simulink model "Firmware"  (R2024b)
settings: Solver=FixedStepDiscrete  StartTime=0.0  StopTime=34.5  FixedStep=0.001  RelTol=1e-3  EnableMultiTasking=on
PreLoadFcn:
  | startup;
  | createVariables;
undefined symbols (not defined in the file or in its folder): B, diff, eour6dof, ESP32, Levenberg, Marquardt, maxWaypoints, Spline, ts, waypointTimes, WROOM, X, Y, Z
libraries: sm_lib x46, nesl_utility x13, blocksLibrary x10, arduinolib x6, simulink_extras x6, robotcorelib x4, robotmaniplib x1, simulink x1
(part 1 of 2)
settings Model: PacingRate=10  ExtModeTrigDuration=2  Creator=esaro  LastModifiedBy=esaro
settings SolverCC: AutoInsertRateTranBlk=on
settings OptimizationCC: EnhancedBackFolding=on  PassReuseOutputArgsAs=Individual arguments  ZeroExternalMemoryAtStartup=off  ZeroInternalMemoryAtStartup=off  MaxStackSize=64  OptimizeBlockOrder=speed  DifferentSizesBufferReuse=on  OptimizationCustomize=off  EfficientTunableParamExpr=on
settings DebuggingCC: ParameterTunabilityLossMsg=error
settings HardwareCC: ProdBitPerPointer=32  ProdBitPerSizeT=32  ProdBitPerPtrDiffT=32  ProdLargestAtomicInteger=Long  ProdLargestAtomicFloat=Double  ProdWordSize=32  ProdHWDeviceType=ARM Compatible->ARM Cortex
settings SFSimCC: MATLABDynamicMemAlloc=off
settings RTWCC: Description=Embedded Coder  SystemTargetFile=ert.tlc  HardwareBoard=ESP32-WROOM(Arduino Compatible)  TLCOptions="-aInlineSetEventsForThisBaseRateFcn=TLC_FALSE -aSuppressMultiTaskScheduler=TLC_FALSE  -aRateBasedStepFcn=0"  TemplateMakefile=ert_default_tmf  Toolchain=ESP32  BuildConfiguration=Faster Runs
settings CodeAppCC: ForceParamTrailComments=on  IgnoreCustomStorageClasses=off  OperatorAnnotations=on  SimulinkDataObjDesc=on  SFDataObjDesc=on  InsertBlockDesc=on
settings ERTTargetCC: SupportContinuousTime=on  SupportVariableSizeSignals=on  ExtModeTransport=3  ExtModeStaticAlloc=on  ExtModeAutomaticAllocSize=off  ExtModeStaticAllocSize=65536  ExtModeMexFile=ext_xcp  ExtModeIntrfLevel=Level2 - Open  InlinedParameterPlacement=Hierarchical

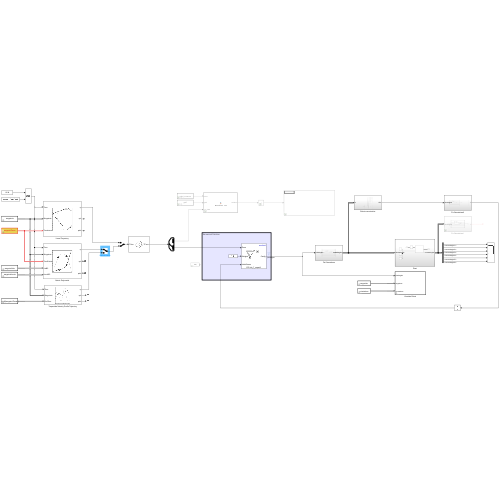
[thumbnail: Simulink's stored preview of the top-level diagram]
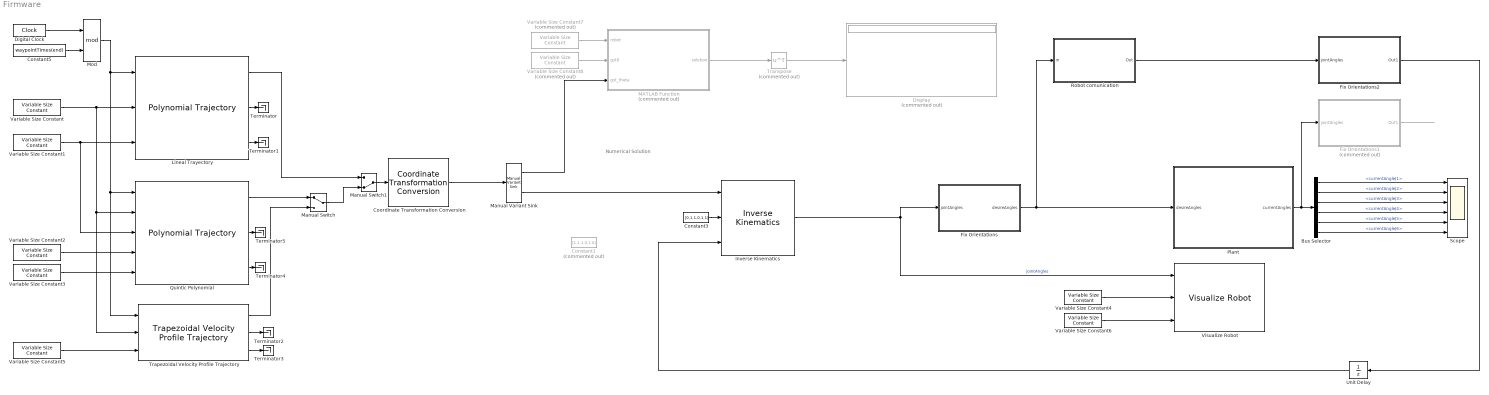
== system Firmware ==
  note: Numerical Solution
  Bus Selector : BusSelector  OutputSignals=currentAngleJ1,currentAngleJ2,currentAngleJ3,currentAngleJ4,currentAngleJ5,currentAngleJ6
  Constant1 : Constant  Commented=on  Value=[1,1,1,0,1,0]  VectorParams1D=off
  Constant3 : Constant  Value=[0,1,1,0,1,1]  VectorParams1D=off
  Constant5 : Constant  Value=waypointTimes(end)
  Coordinate Transformation Conversion : robotcorelib/Coordinate Transformation Conversion  InputRepresentation=Translation Vector  InputEulerSequence=ZYX  ShowTrVecInputPort=on  OutputRepresentation=Homogeneous Transformation  OutputEulerSequence=ZYX  ShowTrVecOutputPort=on  SimulateUsing=Interpreted execution
  Digital Clock : DigitalClock  SampleTime=ts
  Display : Display  Commented=on
  Fix Orientations : Subsystem
  Fix Orientations1 : Subsystem  Commented=on
  Fix Orientations2 : Subsystem
  Inverse Kinematics : robotmaniplib/Inverse Kinematics  RigidBodyTree=eour6dof  EndEffector=link_7_export2  ShowInfo=off  SolverName=Levenberg-Marquardt  EnforceJointLimits=on  MaxIterations=1500  MaxTime=10  GradientTolerance=1e-7  SolutionTolerance=1e-6  StepTolerance=1e-14  ErrorChangeTolerance=1e-12  UseErrorDamping=on  DampingBias=0.0025  SimulateUsing=Interpreted execution
  Lineal Trayectory : robotcorelib/Polynomial Trajectory  WaypointSource=External  Waypoints=[ 0, 2, 1, 5, 0; -1, 3, 1, 4, 4 ]  TimePoints=[ 0, 1, 2, 3, 4 ]  TimeInterval=[ 1, 4 ]  Method=B-Spline  ParameterSource=External  VelocityBoundaryCondition=zeros( 2, 5 )  AccelerationBoundaryCondition=zeros( 2, 5 )  SimulateUsing=Interpreted execution
  MATLAB Function : MATLAB Function  Commented=on  TreatAsAtomicUnit=on
  Manual Variant Sink : simulink/Signal Routing/Manual Variant Sink  NumChoices=2  LabelModeActiveChoice=V_2
  Manual Switch : ManualSwitch
  Manual Switch1 : ManualSwitch  CurrentSetting=0
  Mod : Math  Operator=mod  SignedPower=on
  Plant : Subsystem
  Quintic Polynomial : robotcorelib/Polynomial Trajectory  WaypointSource=External  Waypoints=[ 0, 2, 1, 5, 0; -1, 3, 1, 4, 4 ]  TimePoints=[ 0, 1, 2, 3, 4 ]  TimeInterval=[ 1, 4 ]  Method=Quintic Polynomial  ParameterSource=External  VelocityBoundaryCondition=zeros( 2, 5 )  AccelerationBoundaryCondition=zeros( 2, 5 )  SimulateUsing=Interpreted execution
  Robot comunication : Subsystem
  Scope : Scope  NumInputPorts=6
  Terminator{,1..5} (6 alike) : Terminator
  Transpose : Math  Commented=on  Operator=transpose
  Trapezoidal Velocity Profile Trajectory : robotcorelib/Trapezoidal Velocity Profile Trajectory  WaypointSource=External  Waypoints=[ 0, -0.5, -1; 0, 0.5, 1 ]  NumParams=1  Parameter1=End Time  Parameter2=End Time  ParameterSource=External  PeakVelocity=[ 1; 1; 1 ]  Acceleration=[ 1; 2 ]  EndTime=[ 1; 1; 1 ]  AccelTime=[ 1; 2 ]  SimulateUsing=Interpreted execution
  Unit Delay : UnitDelay  InitialCondition=ikInitGuess'  SampleTime=-1  HasFrameUpgradeWarning=on
  Variable Size Constant : blocksLibrary/Variable Size Constant  val=waypoints  maxSize=[3,maxWaypoints]  Ts=-1
  Variable Size Constant1 : blocksLibrary/Variable Size Constant  val=waypointTimes  maxSize=[1,maxWaypoints]  Ts=-1
  Variable Size Constant2 : blocksLibrary/Variable Size Constant  val=waypointVels  maxSize=[3,maxWaypoints]  Ts=-1
  Variable Size Constant3 : blocksLibrary/Variable Size Constant  val=waypointAccels  maxSize=[3,maxWaypoints]  Ts=-1
  Variable Size Constant4 : blocksLibrary/Variable Size Constant  val=waypoints  maxSize=[3,maxWaypoints]  Ts=-1
  Variable Size Constant5 : blocksLibrary/Variable Size Constant  val=repmat(diff(waypointTimes),[3 1])  maxSize=[3,maxWaypoints-1]  Ts=-1
  Variable Size Constant6 : blocksLibrary/Variable Size Constant  val=orientations  maxSize=[3,maxWaypoints]  Ts=-1
  Variable Size Constant7 : blocksLibrary/Variable Size Constant  Commented=on  val=robot_measure  maxSize=[4,1]  Ts=-1
  Variable Size Constant8 : blocksLibrary/Variable Size Constant  Commented=on  val=gst0  maxSize=[4,4]  Ts=-1
  Visualize Robot : blocksLibrary/Visualize Robot  rbtName=eour6dof  eeName=link_7_export2  numJoints=numel(eour6dof.homeConfiguration)  maxPts=maxWaypoints  plotMode=Trajectory
  wires:
  Bus Selector/1 -> Scope/1  "<currentAngleJ1>"
  Plant/1(currentAngles) -> Fix Orientations1/1(jointAngles), Bus Selector/1
  Constant3/1 -> Inverse Kinematics/2
  Bus Selector/4 -> Scope/4  "<currentAngleJ4>"
  Bus Selector/5 -> Scope/5  "<currentAngleJ5>"
  Bus Selector/6 -> Scope/6  "<currentAngleJ6>"
  Unit Delay/1 -> Inverse Kinematics/3
  Bus Selector/2 -> Scope/2  "<currentAngleJ2>"
  Digital Clock/1 -> Mod/1
  Constant5/1 -> Mod/2
  Trapezoidal Velocity Profile Trajectory/1 -> Manual Switch/2
  Trapezoidal Velocity Profile Trajectory/2 -> Terminator2/1
  Variable Size Constant3/1 -> Quintic Polynomial/5
  Variable Size Constant5/1 -> Trapezoidal Velocity Profile Trajectory/3
  Variable Size Constant2/1 -> Quintic Polynomial/4
  Lineal Trayectory/2 -> Terminator/1
  Trapezoidal Velocity Profile Trajectory/3 -> Terminator3/1
  Lineal Trayectory/3 -> Terminator1/1
  Variable Size Constant6/1 -> Visualize Robot/3
  Manual Switch1/1 -> Coordinate Transformation Conversion/1
  Manual Switch/1 -> Manual Switch1/2
  Lineal Trayectory/1 -> Manual Switch1/1
  Quintic Polynomial/3 -> Terminator4/1
  Quintic Polynomial/2 -> Terminator5/1
  Quintic Polynomial/1 -> Manual Switch/1
  Bus Selector/3 -> Scope/3  "<currentAngleJ3>"
  Robot comunication/1(Out) -> Fix Orientations2/1(jointAngles)
  Fix Orientations/1(desireAngles) -> Plant/1(desireAngles), Robot comunication/1(in)
  Fix Orientations1/1(Out1) -> ?
  Fix Orientations2/1(Out1) -> Unit Delay/1
  Mod/1 -> Lineal Trayectory/1, Trapezoidal Velocity Profile Trajectory/1, Quintic Polynomial/1
  Inverse Kinematics/1 -> Fix Orientations/1(jointAngles), Visualize Robot/1  "jointAngles"
  Variable Size Constant/1 -> Lineal Trayectory/2, Quintic Polynomial/2, Trapezoidal Velocity Profile Trajectory/2
  Variable Size Constant1/1 -> Lineal Trayectory/3, Quintic Polynomial/3
  Variable Size Constant4/1 -> Visualize Robot/2
  Coordinate Transformation Conversion/1 -> Manual Variant Sink/1
  Manual Variant Sink/2 -> Inverse Kinematics/1
  Manual Variant Sink/1 -> MATLAB Function/3(gst_theta)
  MATLAB Function/1(solution) -> Transpose/1
  Transpose/1 -> Display/1
  Variable Size Constant7/1 -> MATLAB Function/1(robot)
  Variable Size Constant8/1 -> MATLAB Function/2(gst0)

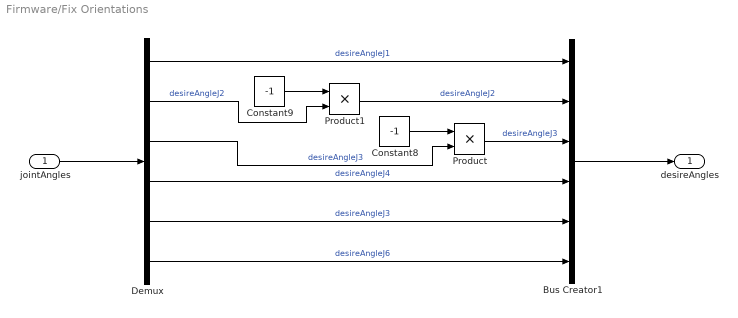
== system Firmware/Fix Orientations ==
  jointAngles : Inport
  Bus Creator1 : BusCreator  Inputs=6
  Constant8 : Constant  Value=-1
  Constant9 : Constant  Value=-1
  Demux : Demux  Outputs=6
  Product : Product
  Product1 : Product
  desireAngles : Outport
  wires:
  Product/1 -> Bus Creator1/3  "desireAngleJ3"
  Product1/1 -> Bus Creator1/2  "desireAngleJ2"
  Constant9/1 -> Product1/1
  Constant8/1 -> Product/1
  Demux/4 -> Bus Creator1/4  "desireAngleJ4"
  Demux/2 -> Product1/2  "desireAngleJ2"
  jointAngles/1 -> Demux/1
  Demux/6 -> Bus Creator1/6  "desireAngleJ6"
  Demux/3 -> Product/2  "desireAngleJ3"
  Demux/1 -> Bus Creator1/1  "desireAngleJ1"
  Bus Creator1/1 -> desireAngles/1
  Demux/5 -> Bus Creator1/5  "desireAngleJ3"

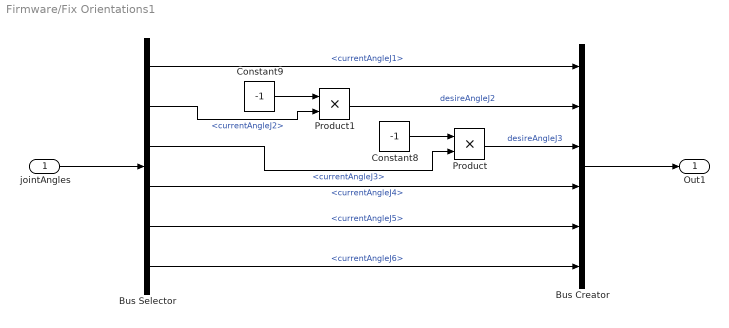
== system Firmware/Fix Orientations1 ==
  jointAngles : Inport
  Bus Creator : BusCreator  Inputs=6
  Bus Selector : BusSelector  OutputSignals=currentAngleJ1,currentAngleJ2,currentAngleJ3,currentAngleJ4,currentAngleJ5,currentAngleJ6
  Constant8 : Constant  Value=-1
  Constant9 : Constant  Value=-1
  Product : Product
  Product1 : Product
  Out1 : Outport
  wires:
  Bus Creator/1 -> Out1/1
  Bus Selector/1 -> Bus Creator/1  "<currentAngleJ1>"
  Bus Selector/3 -> Product/2  "<currentAngleJ3>"
  Bus Selector/6 -> Bus Creator/6  "<currentAngleJ6>"
  Bus Selector/5 -> Bus Creator/5  "<currentAngleJ5>"
  jointAngles/1 -> Bus Selector/1
  Bus Selector/2 -> Product1/2  "<currentAngleJ2>"
  Bus Selector/4 -> Bus Creator/4  "<currentAngleJ4>"
  Constant8/1 -> Product/1
  Constant9/1 -> Product1/1
  Product1/1 -> Bus Creator/2  "desireAngleJ2"
  Product/1 -> Bus Creator/3  "desireAngleJ3"

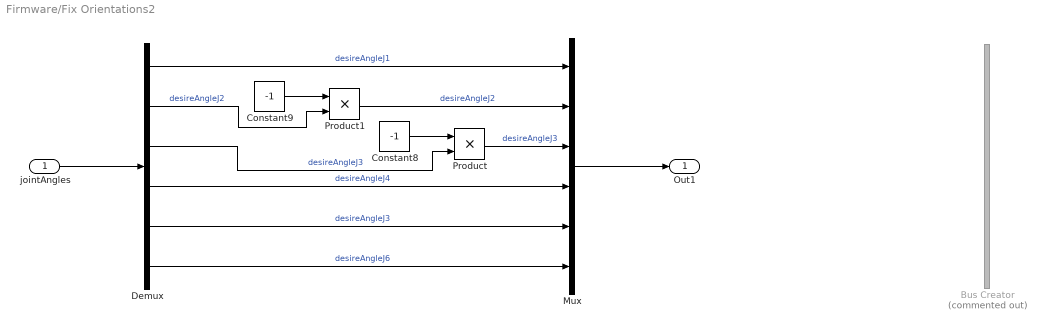
== system Firmware/Fix Orientations2 ==
  jointAngles : Inport
  Bus Creator : BusCreator  Commented=on  Inputs=6
  Constant8 : Constant  Value=-1
  Constant9 : Constant  Value=-1
  Demux : Demux  Outputs=6
  Mux : Mux  Inputs=6
  Product : Product
  Product1 : Product
  Out1 : Outport
  wires:
  Mux/1 -> Out1/1
  Demux/1 -> Mux/1  "desireAngleJ1"
  Demux/3 -> Product/2  "desireAngleJ3"
  Demux/6 -> Mux/6  "desireAngleJ6"
  jointAngles/1 -> Demux/1
  Demux/2 -> Product1/2  "desireAngleJ2"
  Demux/4 -> Mux/4  "desireAngleJ4"
  Constant8/1 -> Product/1
  Constant9/1 -> Product1/1
  Product1/1 -> Mux/2  "desireAngleJ2"
  Product/1 -> Mux/3  "desireAngleJ3"
  Demux/5 -> Mux/5  "desireAngleJ3"

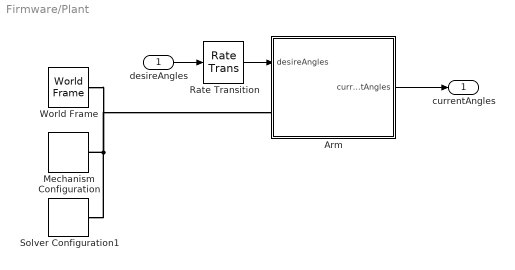
== system Firmware/Plant ==
  desireAngles : Inport
  Arm : Subsystem
  Mechanism Configuration : sm_lib/Utilities/Mechanism Configuration  UniformGravity=Constant  GravityVector=[0 0 -9.80665]  GravityVectorUnits=m/s^2  LinearizationDelta=0.001  JointModeTransitionNonlinearIterations=2
  Rate Transition : RateTransition
  Solver Configuration1 : nesl_utility/Solver Configuration  PhysicalDomain=network_engine_domain  SubClassName=solver  LeftPortType=input  RightPortType=generic  Tones=[]  Harmonics=[]  SimulateNoise=off  Profile=off  UseLocalSampling=off  EnableSwitchedLinearOptims=on  FrequencyDomain=off  UseCCode=off  RelTol=0.001  AbsTol=0.001  MinStep=1e-09  ToWorkspace=off  RevertToSquareIcSolve=off  NumHomotopyIterations=100  PhasorMode=off  PhasorModeNumHarmonics=1  ConsistencySolver=NEWTON_XTOL_AFTER_FTOL  IndexReductionMethod=DerivativeReplacement  DoDC=off  ResidualTolerance=1e-09  ConsistencyTolSource=GLOBAL  ConsistencyAbsTol=0.001  ConsistencyRelTol=0.001  ConsistencyTolFactor=0.5  UseLocalSolver=off  LocalSolverChoice=NE_BACKWARD_EULER_ADVANCER  ResolveIndetEquations=on  FunctionEvalNumThread=1  LocalSolverSampleTime=0.001  DoFixedCost=off  MaxNonlinIter=3  MaxModeIter=2  ComputeImpulses=off  ImpulseIterations=2  LinearAlgebra=auto  LinearAlgebraNumThread=0  EquationFormulation=NE_TIME_EF  DelaysMemoryBudget=1024  AutomaticFiltering=on  FilteringTimeConstant=0.001  PartitionStorageMethod=AS_NEEDED  PartitionMemoryBudget=1024  PartitionMethod=ROBUST  MultibodyUseLocalSolver=off  MultibodyLocalSolverChoice=ODE1  MultibodyLocalSolverSampleTime=0.001
  World Frame : sm_lib/Frames and Transforms/World Frame
  currentAngles : Outport
  wires:
  Arm/1(currentAngles) -> currentAngles/1
  desireAngles/1 -> Rate Transition/1
  Rate Transition/1 -> Arm/1(desireAngles)
  connections:
  Mechanism Configuration/RConn1 -- World Frame/RConn1 -- Arm/LConn1 -- Solver Configuration1/RConn1

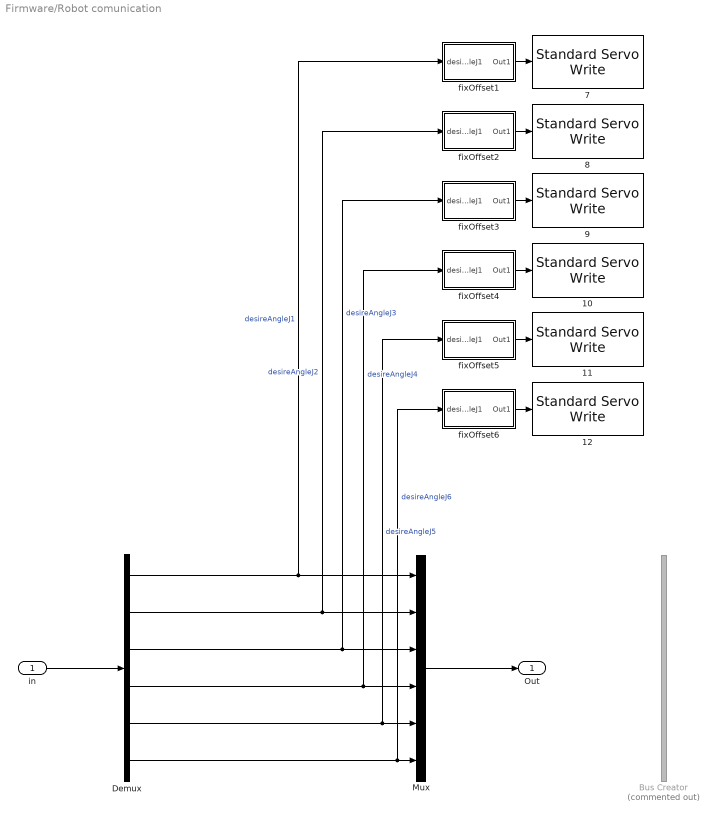
== system Firmware/Robot comunication ==
  in : Inport
  10 : arduinolib/Standard Servo Write  pinNumber=27  ServoIndex=0  blockPlatform=ESP32-WROOM
  11 : arduinolib/Standard Servo Write  pinNumber=14  ServoIndex=1  blockPlatform=ESP32-WROOM
  12 : arduinolib/Standard Servo Write  pinNumber=12  ServoIndex=2  blockPlatform=ESP32-WROOM
  7 : arduinolib/Standard Servo Write  pinNumber=33  ServoIndex=3  blockPlatform=ESP32-WROOM
  8 : arduinolib/Standard Servo Write  pinNumber=25  ServoIndex=4  blockPlatform=ESP32-WROOM
  9 : arduinolib/Standard Servo Write  pinNumber=26  ServoIndex=5  blockPlatform=ESP32-WROOM
  Bus Creator : BusCreator  Commented=on  Inputs=6
  Demux : Demux  Outputs=6
  Mux : Mux  Inputs=6
  fixOffset1 : Subsystem
  fixOffset2 : Subsystem
  fixOffset3 : Subsystem
  fixOffset4 : Subsystem
  fixOffset5 : Subsystem
  fixOffset6 : Subsystem
  Out : Outport
  wires:
  Mux/1 -> Out/1
  fixOffset1/1(Out1) -> 7/1
  Demux/1 -> Mux/1, fixOffset1/1(desireAngleJ1)  "desireAngleJ1"
  Demux/6 -> Mux/6, fixOffset6/1(desireAngleJ1)  "desireAngleJ6"
  Demux/5 -> Mux/5, fixOffset5/1(desireAngleJ1)  "desireAngleJ5"
  in/1 -> Demux/1
  Demux/4 -> Mux/4, fixOffset4/1(desireAngleJ1)  "desireAngleJ4"
  fixOffset2/1(Out1) -> 8/1
  fixOffset4/1(Out1) -> 10/1
  fixOffset3/1(Out1) -> 9/1
  fixOffset6/1(Out1) -> 12/1
  fixOffset5/1(Out1) -> 11/1
  Demux/2 -> Mux/2, fixOffset2/1(desireAngleJ1)  "desireAngleJ2"
  Demux/3 -> Mux/3, fixOffset3/1(desireAngleJ1)  "desireAngleJ3"

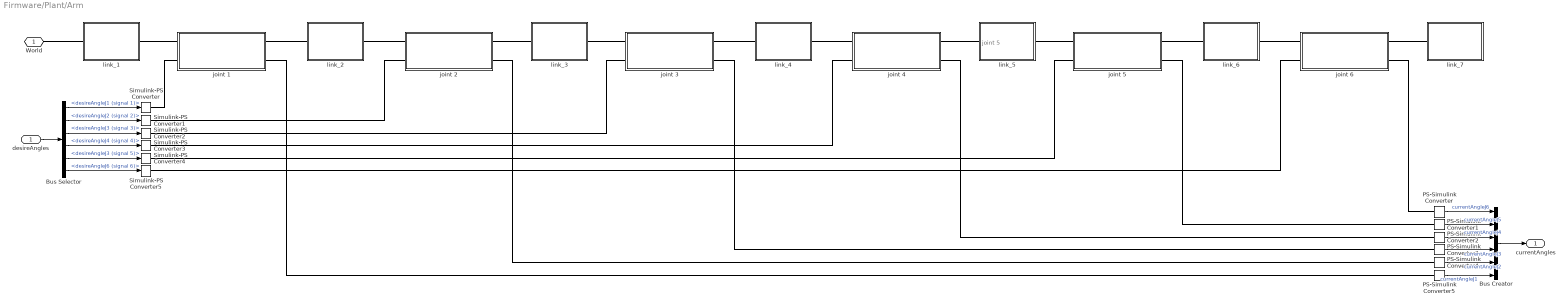
== system Firmware/Plant/Arm ==
  note: joint 5
  desireAngles : Inport
  Bus Creator : BusCreator  Inputs=6
  Bus Selector : BusSelector  OutputSignals=desireAngleJ1 (signal 1),desireAngleJ2 (signal 2),desireAngleJ3 (signal 3),desireAngleJ4 (signal 4),desireAngleJ3 (signal 5),desireAngleJ6 (signal 6)
  PS-Simulink Converter{,1..5} (6 alike) : nesl_utility/PS-Simulink Converter  PhysicalDomain=network_engine_domain  SubClassName=ps_output  LeftPortType=input  RightPortType=output  PseudoPeriodic=off  Frequencies=[]  VectorFormat=inherit  Unit=inherit  AffineConversion=off
  Simulink-PS Converter{,1..5} (6 alike) : nesl_utility/Simulink-PS Converter  PhysicalDomain=network_engine_domain  SubClassName=ps_input  LeftPortType=input  RightPortType=output  PseudoPeriodic=off  Frequencies=[]  NoiseDistribution=none  NoiseParameters=[]  Unit=1  AffineConversion=off  FilteringAndDerivatives=zero  SimscapeFilterOrder=1  InputFilterTimeConstant=0.001  UdotUserProvided=0
  joint 1 : Subsystem
  joint 2 : Subsystem
  joint 3 : Subsystem
  joint 4 : Subsystem
  joint 5 : Subsystem
  joint 6 : Subsystem
  link_1 : Subsystem
  link_2 : Subsystem
  link_3 : Subsystem
  link_4 : Subsystem
  link_5 : Subsystem
  link_6 : Subsystem
  link_7 : Subsystem
  World : PMIOPort  Side=Left
  currentAngles : Outport
  wires:
  Bus Creator/1 -> currentAngles/1
  PS-Simulink Converter/1 -> Bus Creator/1  "currentAngleJ6"
  PS-Simulink Converter1/1 -> Bus Creator/2  "currentAngleJ5"
  PS-Simulink Converter2/1 -> Bus Creator/3  "currentAngleJ4"
  PS-Simulink Converter3/1 -> Bus Creator/4  "currentAngleJ3"
  PS-Simulink Converter4/1 -> Bus Creator/5  "currentAngleJ2"
  PS-Simulink Converter5/1 -> Bus Creator/6  "currentAngleJ1"
  desireAngles/1 -> Bus Selector/1
  Bus Selector/1 -> Simulink-PS Converter/1  "<desireAngleJ1 (signal 1)>"
  Bus Selector/2 -> Simulink-PS Converter1/1  "<desireAngleJ2 (signal 2)>"
  Bus Selector/3 -> Simulink-PS Converter2/1  "<desireAngleJ3 (signal 3)>"
  Bus Selector/4 -> Simulink-PS Converter3/1  "<desireAngleJ4 (signal 4)>"
  Bus Selector/5 -> Simulink-PS Converter4/1  "<desireAngleJ3 (signal 5)>"
  Bus Selector/6 -> Simulink-PS Converter5/1  "<desireAngleJ6 (signal 6)>"
  connections:
  World/RConn1 -- link_1/LConn1
  joint 1/LConn1 -- link_1/RConn1
  joint 1/RConn1 -- link_2/LConn1
  joint 2/LConn1 -- link_2/RConn1
  joint 2/RConn1 -- link_3/LConn1
  joint 3/LConn1 -- link_3/RConn1
  joint 3/RConn1 -- link_4/LConn1
  joint 4/LConn1 -- link_4/RConn1
  joint 4/RConn1 -- link_5/LConn1
  link_5/RConn1 -- joint 5/LConn1
  joint 5/RConn1 -- link_6/LConn1
  link_6/RConn1 -- joint 6/LConn1
  joint 6/RConn1 -- link_7/LConn1
  PS-Simulink Converter/LConn1 -- joint 6/RConn2
  PS-Simulink Converter1/LConn1 -- joint 5/RConn2
  PS-Simulink Converter2/LConn1 -- joint 4/RConn2
  PS-Simulink Converter3/LConn1 -- joint 3/RConn2
  PS-Simulink Converter4/LConn1 -- joint 2/RConn2
  PS-Simulink Converter5/LConn1 -- joint 1/RConn2
  Simulink-PS Converter/RConn1 -- joint 1/LConn2
  Simulink-PS Converter1/RConn1 -- joint 2/LConn2
  Simulink-PS Converter2/RConn1 -- joint 3/LConn2
  Simulink-PS Converter3/RConn1 -- joint 4/LConn2
  Simulink-PS Converter4/RConn1 -- joint 5/LConn2
  joint 6/LConn2 -- Simulink-PS Converter5/RConn1

== system Firmware/Robot comunication/fixOffset1 ==
  desireAngleJ1 : Inport
  Constant2 : Constant  Value=90
  Radians to Degrees : simulink_extras/Transformations/Radians to Degrees
  Sum : Sum  Inputs=|++
  Out1 : Outport
  wires:
  Sum/1 -> Out1/1
  Radians to Degrees/1 -> Sum/1
  desireAngleJ1/1 -> Radians to Degrees/1
  Constant2/1 -> Sum/2

== system Firmware/Robot comunication/fixOffset2 ==
  desireAngleJ1 : Inport
  Constant2 : Constant  Value=90
  Radians to Degrees : simulink_extras/Transformations/Radians to Degrees
  Sum : Sum  Inputs=|++
  Out1 : Outport
  wires:
  Constant2/1 -> Sum/2
  desireAngleJ1/1 -> Radians to Degrees/1
  Radians to Degrees/1 -> Sum/1
  Sum/1 -> Out1/1

== system Firmware/Robot comunication/fixOffset3 ==
  desireAngleJ1 : Inport
  Constant2 : Constant  Value=90
  Radians to Degrees : simulink_extras/Transformations/Radians to Degrees
  Sum : Sum  Inputs=|++
  Out1 : Outport
  wires:
  Sum/1 -> Out1/1
  Radians to Degrees/1 -> Sum/1
  desireAngleJ1/1 -> Radians to Degrees/1
  Constant2/1 -> Sum/2

== system Firmware/Robot comunication/fixOffset4 ==
  desireAngleJ1 : Inport
  Constant2 : Constant  Value=90
  Radians to Degrees : simulink_extras/Transformations/Radians to Degrees
  Sum : Sum  Inputs=|++
  Out1 : Outport
  wires:
  Constant2/1 -> Sum/2
  desireAngleJ1/1 -> Radians to Degrees/1
  Radians to Degrees/1 -> Sum/1
  Sum/1 -> Out1/1

== system Firmware/Robot comunication/fixOffset5 ==
  desireAngleJ1 : Inport
  Constant2 : Constant  Value=90
  Radians to Degrees : simulink_extras/Transformations/Radians to Degrees
  Sum : Sum  Inputs=|++
  Out1 : Outport
  wires:
  Sum/1 -> Out1/1
  Radians to Degrees/1 -> Sum/1
  desireAngleJ1/1 -> Radians to Degrees/1
  Constant2/1 -> Sum/2

== system Firmware/Robot comunication/fixOffset6 ==
  desireAngleJ1 : Inport
  Constant2 : Constant  Value=90
  Radians to Degrees : simulink_extras/Transformations/Radians to Degrees
  Sum : Sum  Inputs=|++
  Out1 : Outport
  wires:
  Constant2/1 -> Sum/2
  desireAngleJ1/1 -> Radians to Degrees/1
  Radians to Degrees/1 -> Sum/1
  Sum/1 -> Out1/1

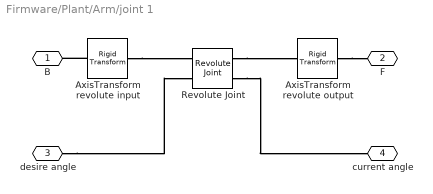
== system Firmware/Plant/Arm/joint 1 ==
  AxisTransform revolute input : sm_lib/Frames and Transforms/Rigid Transform  RotationMethod=ArbitraryAxis  FollAlignAxisA=+X  BaseAlignAxisA=+Y  FollAlignAxisB=+Y  BaseAlignAxisB=+Z  RotationStandardAxis=+Z  RotationAngle=0  RotationAngleUnits=deg  RotationArbitraryAxis=[1 0 0]  RotationSequenceAxes=FollowerAxes  RotationSequence=XYZ  RotationSequenceAngles=[0 0 119.162]  RotationSequenceAnglesUnits=deg  RotationMatrix=[0 0 0; 0 0 0; 0 0 0]  Quaternion=[1 0 0 0]  TranslationMethod=None  TranslationCartesianOffset=[0 0 0]  TranslationCartesianOffsetUnits=m  TranslationStandardAxis=+Z  TranslationStandardOffset=0  TranslationStandardOffsetUnits=m  TranslationROffset=0  TranslationROffsetUnits=m  TranslationThetaOffset=0  TranslationThetaOffsetUnits=deg  TranslationZOffset=0  TranslationZOffsetUnits=m
  AxisTransform revolute output : sm_lib/Frames and Transforms/Rigid Transform  RotationMethod=ArbitraryAxis  FollAlignAxisA=+X  BaseAlignAxisA=+Y  FollAlignAxisB=+Y  BaseAlignAxisB=+Z  RotationStandardAxis=+Z  RotationAngle=0  RotationAngleUnits=deg  RotationArbitraryAxis=[1 0 0]  RotationSequenceAxes=FollowerAxes  RotationSequence=XYZ  RotationSequenceAngles=[0 0 119.162]  RotationSequenceAnglesUnits=deg  RotationMatrix=[0 0 0; 0 0 0; 0 0 0]  Quaternion=[1 0 0 0]  TranslationMethod=None  TranslationCartesianOffset=[0 0 0]  TranslationCartesianOffsetUnits=m  TranslationStandardAxis=+Z  TranslationStandardOffset=0  TranslationStandardOffsetUnits=m  TranslationROffset=0  TranslationROffsetUnits=m  TranslationThetaOffset=0  TranslationThetaOffsetUnits=deg  TranslationZOffset=0  TranslationZOffsetUnits=m
  Revolute Joint : sm_lib/Joints/Revolute Joint  JointMode=Normal  CompositeWrenchDir=FollowerOnBase  CompositeWrenchFrame=BaseFrame  SenseConstraintForce=off  SenseConstraintTorque=off  SenseTotalForce=off  SenseTotalTorque=off  PositionTargetSpecify=off  PositionTargetPriority=High  PositionTargetValue=0  PositionTargetValueUnits=deg  VelocityTargetSpecify=off  VelocityTargetPriority=High  VelocityTargetValue=0  VelocityTargetValueUnits=deg/s  EquilibriumPosition=0  EquilibriumPositionUnits=deg  SpringStiffness=0  SpringStiffnessUnits=N*m/deg  DampingCoefficient=0  DampingCoefficientUnits=N*m/(deg/s)  LowerLimitSpecify=off  LowerLimitBound=-30  LowerLimitBoundUnits=deg  LowerLimitStiffness=1e4  LowerLimitStiffnessUnits=N*m/deg  LowerLimitDamping=10  LowerLimitDampingUnits=N*m/(deg/s)  LowerLimitTransitionRegionWidth=0.1  LowerLimitTransitionRegionWidthUnits=deg  UpperLimitSpecify=off  UpperLimitBound=60  UpperLimitBoundUnits=deg  UpperLimitStiffness=1e4  UpperLimitStiffnessUnits=N*m/deg  UpperLimitDamping=10  UpperLimitDampingUnits=N*m/(deg/s)  UpperLimitTransitionRegionWidth=0.1  UpperLimitTransitionRegionWidthUnits=deg  TorqueActuationMode=ComputedTorque  MotionActuationMode=InputMotion  SensePosition=on  SenseVelocity=off  SenseAcceleration=off  SenseTorqueForce=off  SenseLowerLimitTorqueForce=off  SenseUpperLimitTorqueForce=off
  B : PMIOPort  Side=Left
  F : PMIOPort  Port=2  Side=Right
  desire angle : PMIOPort  Port=3  Side=Left
  current angle : PMIOPort  Port=4  Side=Right
  connections:
  AxisTransform revolute input/LConn1 -- B/RConn1
  AxisTransform revolute input/RConn1 -- Revolute Joint/LConn1
  AxisTransform revolute output/RConn1 -- F/RConn1
  Revolute Joint/RConn1 -- AxisTransform revolute output/LConn1
  desire angle/RConn1 -- Revolute Joint/LConn2
  Revolute Joint/RConn2 -- current angle/RConn1

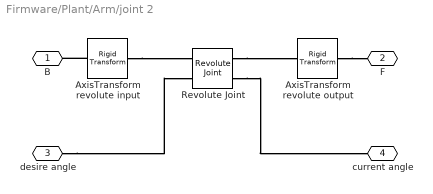
== system Firmware/Plant/Arm/joint 2 ==
  AxisTransform revolute input : sm_lib/Frames and Transforms/Rigid Transform  RotationMethod=ArbitraryAxis  FollAlignAxisA=+X  BaseAlignAxisA=+Y  FollAlignAxisB=+Y  BaseAlignAxisB=+Z  RotationStandardAxis=+Z  RotationAngle=0  RotationAngleUnits=deg  RotationArbitraryAxis=[1 0 0]  RotationSequenceAxes=FollowerAxes  RotationSequence=XYZ  RotationSequenceAngles=[0 0 119.162]  RotationSequenceAnglesUnits=deg  RotationMatrix=[0 0 0; 0 0 0; 0 0 0]  Quaternion=[1 0 0 0]  TranslationMethod=None  TranslationCartesianOffset=[0 0 0]  TranslationCartesianOffsetUnits=m  TranslationStandardAxis=+Z  TranslationStandardOffset=0  TranslationStandardOffsetUnits=m  TranslationROffset=0  TranslationROffsetUnits=m  TranslationThetaOffset=0  TranslationThetaOffsetUnits=deg  TranslationZOffset=0  TranslationZOffsetUnits=m
  AxisTransform revolute output : sm_lib/Frames and Transforms/Rigid Transform  RotationMethod=ArbitraryAxis  FollAlignAxisA=+X  BaseAlignAxisA=+Y  FollAlignAxisB=+Y  BaseAlignAxisB=+Z  RotationStandardAxis=+Z  RotationAngle=0  RotationAngleUnits=deg  RotationArbitraryAxis=[1 0 0]  RotationSequenceAxes=FollowerAxes  RotationSequence=XYZ  RotationSequenceAngles=[0 0 119.162]  RotationSequenceAnglesUnits=deg  RotationMatrix=[0 0 0; 0 0 0; 0 0 0]  Quaternion=[1 0 0 0]  TranslationMethod=None  TranslationCartesianOffset=[0 0 0]  TranslationCartesianOffsetUnits=m  TranslationStandardAxis=+Z  TranslationStandardOffset=0  TranslationStandardOffsetUnits=m  TranslationROffset=0  TranslationROffsetUnits=m  TranslationThetaOffset=0  TranslationThetaOffsetUnits=deg  TranslationZOffset=0  TranslationZOffsetUnits=m
  Revolute Joint : sm_lib/Joints/Revolute Joint  JointMode=Normal  CompositeWrenchDir=FollowerOnBase  CompositeWrenchFrame=BaseFrame  SenseConstraintForce=off  SenseConstraintTorque=off  SenseTotalForce=off  SenseTotalTorque=off  PositionTargetSpecify=off  PositionTargetPriority=High  PositionTargetValue=0  PositionTargetValueUnits=deg  VelocityTargetSpecify=off  VelocityTargetPriority=High  VelocityTargetValue=0  VelocityTargetValueUnits=deg/s  EquilibriumPosition=0  EquilibriumPositionUnits=deg  SpringStiffness=0  SpringStiffnessUnits=N*m/deg  DampingCoefficient=0  DampingCoefficientUnits=N*m/(deg/s)  LowerLimitSpecify=off  LowerLimitBound=-30  LowerLimitBoundUnits=deg  LowerLimitStiffness=1e4  LowerLimitStiffnessUnits=N*m/deg  LowerLimitDamping=10  LowerLimitDampingUnits=N*m/(deg/s)  LowerLimitTransitionRegionWidth=0.1  LowerLimitTransitionRegionWidthUnits=deg  UpperLimitSpecify=off  UpperLimitBound=60  UpperLimitBoundUnits=deg  UpperLimitStiffness=1e4  UpperLimitStiffnessUnits=N*m/deg  UpperLimitDamping=10  UpperLimitDampingUnits=N*m/(deg/s)  UpperLimitTransitionRegionWidth=0.1  UpperLimitTransitionRegionWidthUnits=deg  TorqueActuationMode=ComputedTorque  MotionActuationMode=InputMotion  SensePosition=on  SenseVelocity=off  SenseAcceleration=off  SenseTorqueForce=off  SenseLowerLimitTorqueForce=off  SenseUpperLimitTorqueForce=off
  B : PMIOPort  Side=Left
  F : PMIOPort  Port=2  Side=Right
  desire angle : PMIOPort  Port=3  Side=Left
  current angle : PMIOPort  Port=4  Side=Right
  connections:
  AxisTransform revolute input/LConn1 -- B/RConn1
  AxisTransform revolute input/RConn1 -- Revolute Joint/LConn1
  AxisTransform revolute output/RConn1 -- F/RConn1
  Revolute Joint/RConn1 -- AxisTransform revolute output/LConn1
  desire angle/RConn1 -- Revolute Joint/LConn2
  Revolute Joint/RConn2 -- current angle/RConn1

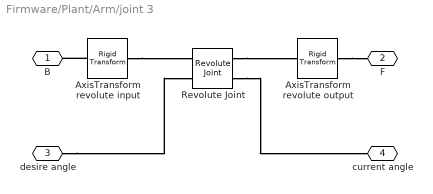
== system Firmware/Plant/Arm/joint 3 ==
  AxisTransform revolute input : sm_lib/Frames and Transforms/Rigid Transform  RotationMethod=ArbitraryAxis  FollAlignAxisA=+X  BaseAlignAxisA=+Y  FollAlignAxisB=+Y  BaseAlignAxisB=+Z  RotationStandardAxis=+Z  RotationAngle=0  RotationAngleUnits=deg  RotationArbitraryAxis=[1 0 0]  RotationSequenceAxes=FollowerAxes  RotationSequence=XYZ  RotationSequenceAngles=[0 0 119.162]  RotationSequenceAnglesUnits=deg  RotationMatrix=[0 0 0; 0 0 0; 0 0 0]  Quaternion=[1 0 0 0]  TranslationMethod=None  TranslationCartesianOffset=[0 0 0]  TranslationCartesianOffsetUnits=m  TranslationStandardAxis=+Z  TranslationStandardOffset=0  TranslationStandardOffsetUnits=m  TranslationROffset=0  TranslationROffsetUnits=m  TranslationThetaOffset=0  TranslationThetaOffsetUnits=deg  TranslationZOffset=0  TranslationZOffsetUnits=m
  AxisTransform revolute output : sm_lib/Frames and Transforms/Rigid Transform  RotationMethod=ArbitraryAxis  FollAlignAxisA=+X  BaseAlignAxisA=+Y  FollAlignAxisB=+Y  BaseAlignAxisB=+Z  RotationStandardAxis=+Z  RotationAngle=0  RotationAngleUnits=deg  RotationArbitraryAxis=[1 0 0]  RotationSequenceAxes=FollowerAxes  RotationSequence=XYZ  RotationSequenceAngles=[0 0 119.162]  RotationSequenceAnglesUnits=deg  RotationMatrix=[0 0 0; 0 0 0; 0 0 0]  Quaternion=[1 0 0 0]  TranslationMethod=None  TranslationCartesianOffset=[0 0 0]  TranslationCartesianOffsetUnits=m  TranslationStandardAxis=+Z  TranslationStandardOffset=0  TranslationStandardOffsetUnits=m  TranslationROffset=0  TranslationROffsetUnits=m  TranslationThetaOffset=0  TranslationThetaOffsetUnits=deg  TranslationZOffset=0  TranslationZOffsetUnits=m
  Revolute Joint : sm_lib/Joints/Revolute Joint  JointMode=Normal  CompositeWrenchDir=FollowerOnBase  CompositeWrenchFrame=BaseFrame  SenseConstraintForce=off  SenseConstraintTorque=off  SenseTotalForce=off  SenseTotalTorque=off  PositionTargetSpecify=off  PositionTargetPriority=High  PositionTargetValue=0  PositionTargetValueUnits=deg  VelocityTargetSpecify=off  VelocityTargetPriority=High  VelocityTargetValue=0  VelocityTargetValueUnits=deg/s  EquilibriumPosition=0  EquilibriumPositionUnits=deg  SpringStiffness=0  SpringStiffnessUnits=N*m/deg  DampingCoefficient=0  DampingCoefficientUnits=N*m/(deg/s)  LowerLimitSpecify=off  LowerLimitBound=-30  LowerLimitBoundUnits=deg  LowerLimitStiffness=1e4  LowerLimitStiffnessUnits=N*m/deg  LowerLimitDamping=10  LowerLimitDampingUnits=N*m/(deg/s)  LowerLimitTransitionRegionWidth=0.1  LowerLimitTransitionRegionWidthUnits=deg  UpperLimitSpecify=off  UpperLimitBound=60  UpperLimitBoundUnits=deg  UpperLimitStiffness=1e4  UpperLimitStiffnessUnits=N*m/deg  UpperLimitDamping=10  UpperLimitDampingUnits=N*m/(deg/s)  UpperLimitTransitionRegionWidth=0.1  UpperLimitTransitionRegionWidthUnits=deg  TorqueActuationMode=ComputedTorque  MotionActuationMode=InputMotion  SensePosition=on  SenseVelocity=off  SenseAcceleration=off  SenseTorqueForce=off  SenseLowerLimitTorqueForce=off  SenseUpperLimitTorqueForce=off
  B : PMIOPort  Side=Left
  F : PMIOPort  Port=2  Side=Right
  desire angle : PMIOPort  Port=3  Side=Left
  current angle : PMIOPort  Port=4  Side=Right
  connections:
  AxisTransform revolute input/LConn1 -- B/RConn1
  AxisTransform revolute input/RConn1 -- Revolute Joint/LConn1
  AxisTransform revolute output/RConn1 -- F/RConn1
  Revolute Joint/RConn1 -- AxisTransform revolute output/LConn1
  desire angle/RConn1 -- Revolute Joint/LConn2
  Revolute Joint/RConn2 -- current angle/RConn1

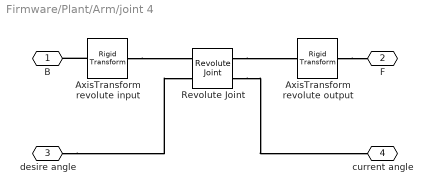
== system Firmware/Plant/Arm/joint 4 ==
  AxisTransform revolute input : sm_lib/Frames and Transforms/Rigid Transform  RotationMethod=ArbitraryAxis  FollAlignAxisA=+X  BaseAlignAxisA=+Y  FollAlignAxisB=+Y  BaseAlignAxisB=+Z  RotationStandardAxis=+Z  RotationAngle=0  RotationAngleUnits=deg  RotationArbitraryAxis=[1 0 0]  RotationSequenceAxes=FollowerAxes  RotationSequence=XYZ  RotationSequenceAngles=[0 0 119.162]  RotationSequenceAnglesUnits=deg  RotationMatrix=[0 0 0; 0 0 0; 0 0 0]  Quaternion=[1 0 0 0]  TranslationMethod=None  TranslationCartesianOffset=[0 0 0]  TranslationCartesianOffsetUnits=m  TranslationStandardAxis=+Z  TranslationStandardOffset=0  TranslationStandardOffsetUnits=m  TranslationROffset=0  TranslationROffsetUnits=m  TranslationThetaOffset=0  TranslationThetaOffsetUnits=deg  TranslationZOffset=0  TranslationZOffsetUnits=m
  AxisTransform revolute output : sm_lib/Frames and Transforms/Rigid Transform  RotationMethod=ArbitraryAxis  FollAlignAxisA=+X  BaseAlignAxisA=+Y  FollAlignAxisB=+Y  BaseAlignAxisB=+Z  RotationStandardAxis=+Z  RotationAngle=0  RotationAngleUnits=deg  RotationArbitraryAxis=[1 0 0]  RotationSequenceAxes=FollowerAxes  RotationSequence=XYZ  RotationSequenceAngles=[0 0 119.162]  RotationSequenceAnglesUnits=deg  RotationMatrix=[0 0 0; 0 0 0; 0 0 0]  Quaternion=[1 0 0 0]  TranslationMethod=None  TranslationCartesianOffset=[0 0 0]  TranslationCartesianOffsetUnits=m  TranslationStandardAxis=+Z  TranslationStandardOffset=0  TranslationStandardOffsetUnits=m  TranslationROffset=0  TranslationROffsetUnits=m  TranslationThetaOffset=0  TranslationThetaOffsetUnits=deg  TranslationZOffset=0  TranslationZOffsetUnits=m
  Revolute Joint : sm_lib/Joints/Revolute Joint  JointMode=Normal  CompositeWrenchDir=FollowerOnBase  CompositeWrenchFrame=BaseFrame  SenseConstraintForce=off  SenseConstraintTorque=off  SenseTotalForce=off  SenseTotalTorque=off  PositionTargetSpecify=off  PositionTargetPriority=High  PositionTargetValue=0  PositionTargetValueUnits=deg  VelocityTargetSpecify=off  VelocityTargetPriority=High  VelocityTargetValue=0  VelocityTargetValueUnits=deg/s  EquilibriumPosition=0  EquilibriumPositionUnits=deg  SpringStiffness=0  SpringStiffnessUnits=N*m/deg  DampingCoefficient=0  DampingCoefficientUnits=N*m/(deg/s)  LowerLimitSpecify=off  LowerLimitBound=-30  LowerLimitBoundUnits=deg  LowerLimitStiffness=1e4  LowerLimitStiffnessUnits=N*m/deg  LowerLimitDamping=10  LowerLimitDampingUnits=N*m/(deg/s)  LowerLimitTransitionRegionWidth=0.1  LowerLimitTransitionRegionWidthUnits=deg  UpperLimitSpecify=off  UpperLimitBound=60  UpperLimitBoundUnits=deg  UpperLimitStiffness=1e4  UpperLimitStiffnessUnits=N*m/deg  UpperLimitDamping=10  UpperLimitDampingUnits=N*m/(deg/s)  UpperLimitTransitionRegionWidth=0.1  UpperLimitTransitionRegionWidthUnits=deg  TorqueActuationMode=ComputedTorque  MotionActuationMode=InputMotion  SensePosition=on  SenseVelocity=off  SenseAcceleration=off  SenseTorqueForce=off  SenseLowerLimitTorqueForce=off  SenseUpperLimitTorqueForce=off
  B : PMIOPort  Side=Left
  F : PMIOPort  Port=2  Side=Right
  desire angle : PMIOPort  Port=3  Side=Left
  current angle : PMIOPort  Port=4  Side=Right
  connections:
  AxisTransform revolute input/LConn1 -- B/RConn1
  AxisTransform revolute input/RConn1 -- Revolute Joint/LConn1
  AxisTransform revolute output/RConn1 -- F/RConn1
  Revolute Joint/RConn1 -- AxisTransform revolute output/LConn1
  desire angle/RConn1 -- Revolute Joint/LConn2
  Revolute Joint/RConn2 -- current angle/RConn1

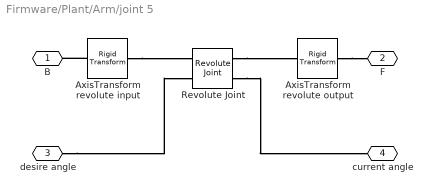
== system Firmware/Plant/Arm/joint 5 ==
  AxisTransform revolute input : sm_lib/Frames and Transforms/Rigid Transform  RotationMethod=ArbitraryAxis  FollAlignAxisA=+X  BaseAlignAxisA=+Y  FollAlignAxisB=+Y  BaseAlignAxisB=+Z  RotationStandardAxis=+Z  RotationAngle=0  RotationAngleUnits=deg  RotationArbitraryAxis=[1 0 0]  RotationSequenceAxes=FollowerAxes  RotationSequence=XYZ  RotationSequenceAngles=[0 0 119.162]  RotationSequenceAnglesUnits=deg  RotationMatrix=[0 0 0; 0 0 0; 0 0 0]  Quaternion=[1 0 0 0]  TranslationMethod=None  TranslationCartesianOffset=[0 0 0]  TranslationCartesianOffsetUnits=m  TranslationStandardAxis=+Z  TranslationStandardOffset=0  TranslationStandardOffsetUnits=m  TranslationROffset=0  TranslationROffsetUnits=m  TranslationThetaOffset=0  TranslationThetaOffsetUnits=deg  TranslationZOffset=0  TranslationZOffsetUnits=m
  AxisTransform revolute output : sm_lib/Frames and Transforms/Rigid Transform  RotationMethod=ArbitraryAxis  FollAlignAxisA=+X  BaseAlignAxisA=+Y  FollAlignAxisB=+Y  BaseAlignAxisB=+Z  RotationStandardAxis=+Z  RotationAngle=0  RotationAngleUnits=deg  RotationArbitraryAxis=[1 0 0]  RotationSequenceAxes=FollowerAxes  RotationSequence=XYZ  RotationSequenceAngles=[0 0 119.162]  RotationSequenceAnglesUnits=deg  RotationMatrix=[0 0 0; 0 0 0; 0 0 0]  Quaternion=[1 0 0 0]  TranslationMethod=None  TranslationCartesianOffset=[0 0 0]  TranslationCartesianOffsetUnits=m  TranslationStandardAxis=+Z  TranslationStandardOffset=0  TranslationStandardOffsetUnits=m  TranslationROffset=0  TranslationROffsetUnits=m  TranslationThetaOffset=0  TranslationThetaOffsetUnits=deg  TranslationZOffset=0  TranslationZOffsetUnits=m
  Revolute Joint : sm_lib/Joints/Revolute Joint  JointMode=Normal  CompositeWrenchDir=FollowerOnBase  CompositeWrenchFrame=BaseFrame  SenseConstraintForce=off  SenseConstraintTorque=off  SenseTotalForce=off  SenseTotalTorque=off  PositionTargetSpecify=off  PositionTargetPriority=High  PositionTargetValue=0  PositionTargetValueUnits=deg  VelocityTargetSpecify=off  VelocityTargetPriority=High  VelocityTargetValue=0  VelocityTargetValueUnits=deg/s  EquilibriumPosition=0  EquilibriumPositionUnits=deg  SpringStiffness=0  SpringStiffnessUnits=N*m/deg  DampingCoefficient=0  DampingCoefficientUnits=N*m/(deg/s)  LowerLimitSpecify=off  LowerLimitBound=-30  LowerLimitBoundUnits=deg  LowerLimitStiffness=1e4  LowerLimitStiffnessUnits=N*m/deg  LowerLimitDamping=10  LowerLimitDampingUnits=N*m/(deg/s)  LowerLimitTransitionRegionWidth=0.1  LowerLimitTransitionRegionWidthUnits=deg  UpperLimitSpecify=off  UpperLimitBound=60  UpperLimitBoundUnits=deg  UpperLimitStiffness=1e4  UpperLimitStiffnessUnits=N*m/deg  UpperLimitDamping=10  UpperLimitDampingUnits=N*m/(deg/s)  UpperLimitTransitionRegionWidth=0.1  UpperLimitTransitionRegionWidthUnits=deg  TorqueActuationMode=ComputedTorque  MotionActuationMode=InputMotion  SensePosition=on  SenseVelocity=off  SenseAcceleration=off  SenseTorqueForce=off  SenseLowerLimitTorqueForce=off  SenseUpperLimitTorqueForce=off
  B : PMIOPort  Side=Left
  F : PMIOPort  Port=2  Side=Right
  desire angle : PMIOPort  Port=3  Side=Left
  current angle : PMIOPort  Port=4  Side=Right
  connections:
  AxisTransform revolute input/LConn1 -- B/RConn1
  AxisTransform revolute input/RConn1 -- Revolute Joint/LConn1
  AxisTransform revolute output/RConn1 -- F/RConn1
  Revolute Joint/RConn1 -- AxisTransform revolute output/LConn1
  desire angle/RConn1 -- Revolute Joint/LConn2
  Revolute Joint/RConn2 -- current angle/RConn1

== system Firmware/Plant/Arm/joint 6 ==
  AxisTransform revolute input : sm_lib/Frames and Transforms/Rigid Transform  RotationMethod=ArbitraryAxis  FollAlignAxisA=+X  BaseAlignAxisA=+Y  FollAlignAxisB=+Y  BaseAlignAxisB=+Z  RotationStandardAxis=+Z  RotationAngle=0  RotationAngleUnits=deg  RotationArbitraryAxis=[1 0 0]  RotationSequenceAxes=FollowerAxes  RotationSequence=XYZ  RotationSequenceAngles=[0 0 119.162]  RotationSequenceAnglesUnits=deg  RotationMatrix=[0 0 0; 0 0 0; 0 0 0]  Quaternion=[1 0 0 0]  TranslationMethod=None  TranslationCartesianOffset=[0 0 0]  TranslationCartesianOffsetUnits=m  TranslationStandardAxis=+Z  TranslationStandardOffset=0  TranslationStandardOffsetUnits=m  TranslationROffset=0  TranslationROffsetUnits=m  TranslationThetaOffset=0  TranslationThetaOffsetUnits=deg  TranslationZOffset=0  TranslationZOffsetUnits=m
  AxisTransform revolute output : sm_lib/Frames and Transforms/Rigid Transform  RotationMethod=ArbitraryAxis  FollAlignAxisA=+X  BaseAlignAxisA=+Y  FollAlignAxisB=+Y  BaseAlignAxisB=+Z  RotationStandardAxis=+Z  RotationAngle=0  RotationAngleUnits=deg  RotationArbitraryAxis=[1 0 0]  RotationSequenceAxes=FollowerAxes  RotationSequence=XYZ  RotationSequenceAngles=[0 0 119.162]  RotationSequenceAnglesUnits=deg  RotationMatrix=[0 0 0; 0 0 0; 0 0 0]  Quaternion=[1 0 0 0]  TranslationMethod=None  TranslationCartesianOffset=[0 0 0]  TranslationCartesianOffsetUnits=m  TranslationStandardAxis=+Z  TranslationStandardOffset=0  TranslationStandardOffsetUnits=m  TranslationROffset=0  TranslationROffsetUnits=m  TranslationThetaOffset=0  TranslationThetaOffsetUnits=deg  TranslationZOffset=0  TranslationZOffsetUnits=m
  Revolute Joint : sm_lib/Joints/Revolute Joint  JointMode=Normal  CompositeWrenchDir=FollowerOnBase  CompositeWrenchFrame=BaseFrame  SenseConstraintForce=off  SenseConstraintTorque=off  SenseTotalForce=off  SenseTotalTorque=off  PositionTargetSpecify=off  PositionTargetPriority=High  PositionTargetValue=0  PositionTargetValueUnits=deg  VelocityTargetSpecify=off  VelocityTargetPriority=High  VelocityTargetValue=0  VelocityTargetValueUnits=deg/s  EquilibriumPosition=0  EquilibriumPositionUnits=deg  SpringStiffness=0  SpringStiffnessUnits=N*m/deg  DampingCoefficient=0  DampingCoefficientUnits=N*m/(deg/s)  LowerLimitSpecify=off  LowerLimitBound=-30  LowerLimitBoundUnits=deg  LowerLimitStiffness=1e4  LowerLimitStiffnessUnits=N*m/deg  LowerLimitDamping=10  LowerLimitDampingUnits=N*m/(deg/s)  LowerLimitTransitionRegionWidth=0.1  LowerLimitTransitionRegionWidthUnits=deg  UpperLimitSpecify=off  UpperLimitBound=60  UpperLimitBoundUnits=deg  UpperLimitStiffness=1e4  UpperLimitStiffnessUnits=N*m/deg  UpperLimitDamping=10  UpperLimitDampingUnits=N*m/(deg/s)  UpperLimitTransitionRegionWidth=0.1  UpperLimitTransitionRegionWidthUnits=deg  TorqueActuationMode=ComputedTorque  MotionActuationMode=InputMotion  SensePosition=on  SenseVelocity=off  SenseAcceleration=off  SenseTorqueForce=off  SenseLowerLimitTorqueForce=off  SenseUpperLimitTorqueForce=off
  B : PMIOPort  Side=Left
  F : PMIOPort  Port=2  Side=Right
  desire angle : PMIOPort  Port=3  Side=Left
  current angle : PMIOPort  Port=4  Side=Right
  connections:
  AxisTransform revolute input/LConn1 -- B/RConn1
  AxisTransform revolute input/RConn1 -- Revolute Joint/LConn1
  AxisTransform revolute output/RConn1 -- F/RConn1
  Revolute Joint/RConn1 -- AxisTransform revolute output/LConn1
  desire angle/RConn1 -- Revolute Joint/LConn2
  Revolute Joint/RConn2 -- current angle/RConn1

== system Firmware/Plant/Arm/link_1 ==
  AxisTransform revolute link_2 : sm_lib/Frames and Transforms/Rigid Transform  RotationMethod=None  FollAlignAxisA=+X  BaseAlignAxisA=+Y  FollAlignAxisB=+Y  BaseAlignAxisB=+Z  RotationStandardAxis=+Z  RotationAngle=0  RotationAngleUnits=deg  RotationArbitraryAxis=[0 0 1]  RotationSequenceAxes=FollowerAxes  RotationSequence=XYZ  RotationSequenceAngles=[0 0 119.162]  RotationSequenceAnglesUnits=deg  RotationMatrix=[0 0 0; 0 0 0; 0 0 0]  Quaternion=[1 0 0 0]  TranslationMethod=None  TranslationCartesianOffset=[0 0 0]  TranslationCartesianOffsetUnits=m  TranslationStandardAxis=+Z  TranslationStandardOffset=0  TranslationStandardOffsetUnits=m  TranslationROffset=0  TranslationROffsetUnits=m  TranslationThetaOffset=0  TranslationThetaOffsetUnits=deg  TranslationZOffset=0  TranslationZOffsetUnits=m
  OriginTransform revolute link_2 : sm_lib/Frames and Transforms/Rigid Transform  RotationMethod=None  FollAlignAxisA=+X  BaseAlignAxisA=+Y  FollAlignAxisB=+Y  BaseAlignAxisB=+Z  RotationStandardAxis=+Z  RotationAngle=0  RotationAngleUnits=deg  RotationArbitraryAxis=[0 0 1]  RotationSequenceAxes=FollowerAxes  RotationSequence=XYX  RotationSequenceAngles=[0 0 0]  RotationSequenceAnglesUnits=deg  RotationMatrix=[1 0 0;0 1 0;0 0 1]  Quaternion=[1 0 0 0]  TranslationMethod=Cartesian  TranslationCartesianOffset=[0 0.00 31.533]  TranslationCartesianOffsetUnits=mm  TranslationStandardAxis=+Z  TranslationStandardOffset=0  TranslationStandardOffsetUnits=m  TranslationROffset=0  TranslationROffsetUnits=m  TranslationThetaOffset=0  TranslationThetaOffsetUnits=deg  TranslationZOffset=0  TranslationZOffsetUnits=m
  Reference Frame : sm_lib/Frames and Transforms/Reference Frame
  link_1 : sm_lib/Body Elements/File Solid  ExtGeomFileName=./meshes/link_1.stl  UnitType=Custom  ExtGeomFileUnits=mm  StepReaderType=HEX  ExportConvexHullGeometry=off  InertiaType=CalculateFromGeometry  BasedOnType=Mass  Density=7986.89  DensityUnits=kg/m^3  Mass=680.695  MassUnits=g  CenterOfMass=[0.00, 0.00, 7.613]  CenterOfMassUnits=mm  MomentsOfInertia=[1 1 1]  MomentsOfInertiaUnits=g*mm^2  ProductsOfInertia=[0 0 0]  ProductsOfInertiaUnits=g*mm^2  GraphicType=FromGeometry  MarkerShape=Sphere  MarkerSize=10  GraphicVisPropType=SimpleVisualProperties  GraphicDiffuseColor=[0.5 0.5 0.5]  GraphicOpacity=1.0  GraphicSpecularColor=[0.5 0.5 0.5 1.0]  GraphicAmbientColor=[0.15 0.15 0.15 1.0]  GraphicEmissiveColor=[0.0 0.0 0.0 1.0]  GraphicShininess=75  DoExposeReferenceFrame=on  SerializedFrames=<Frames/>
  world : PMIOPort  Side=Left
  joint 1 : PMIOPort  Port=2  Side=Right
  connections:
  OriginTransform revolute link_2/LConn1 -- link_1/RConn1 -- world/RConn1 -- Reference Frame/RConn1
  AxisTransform revolute link_2/LConn1 -- OriginTransform revolute link_2/RConn1
  joint 1/RConn1 -- AxisTransform revolute link_2/RConn1

== system Firmware/Plant/Arm/link_2 ==
  AxisTransform revolute link_3 : sm_lib/Frames and Transforms/Rigid Transform  RotationMethod=RotationSequence  FollAlignAxisA=+X  BaseAlignAxisA=+Y  FollAlignAxisB=+Y  BaseAlignAxisB=+Z  RotationStandardAxis=+Z  RotationAngle=0  RotationAngleUnits=deg  RotationArbitraryAxis=[0 0 1]  RotationSequenceAxes=FollowerAxes  RotationSequence=YXZ  RotationSequenceAngles=[-90 180 0]  RotationSequenceAnglesUnits=deg  RotationMatrix=[-1.836970198721030e-16,1,0;-1,-1.836970198721030e-16,0;0,0,1]  Quaternion=[1 0 0 0]  TranslationMethod=None  TranslationCartesianOffset=[0 0 0]  TranslationCartesianOffsetUnits=m  TranslationStandardAxis=+Z  TranslationStandardOffset=0  TranslationStandardOffsetUnits=m  TranslationROffset=0  TranslationROffsetUnits=m  TranslationThetaOffset=0  TranslationThetaOffsetUnits=deg  TranslationZOffset=0  TranslationZOffsetUnits=m
  OriginTransform revolute link_3 : sm_lib/Frames and Transforms/Rigid Transform  RotationMethod=None  FollAlignAxisA=+X  BaseAlignAxisA=+Y  FollAlignAxisB=+Y  BaseAlignAxisB=+Z  RotationStandardAxis=+Z  RotationAngle=0  RotationAngleUnits=deg  RotationArbitraryAxis=[0 0 1]  RotationSequenceAxes=FollowerAxes  RotationSequence=XYX  RotationSequenceAngles=[0 0 0]  RotationSequenceAnglesUnits=deg  RotationMatrix=[1 0 0;0 1 0;0 0 1]  Quaternion=[1 0 0 0]  TranslationMethod=Cartesian  TranslationCartesianOffset=[5.245 0.00 56.18]  TranslationCartesianOffsetUnits=mm  TranslationStandardAxis=+Z  TranslationStandardOffset=0  TranslationStandardOffsetUnits=m  TranslationROffset=0  TranslationROffsetUnits=m  TranslationThetaOffset=0  TranslationThetaOffsetUnits=deg  TranslationZOffset=0  TranslationZOffsetUnits=m
  Reference Frame : sm_lib/Frames and Transforms/Reference Frame
  link_2 : sm_lib/Body Elements/File Solid  ExtGeomFileName=./meshes/link_2.stl  UnitType=Custom  ExtGeomFileUnits=mm  StepReaderType=HEX  ExportConvexHullGeometry=off  InertiaType=CalculateFromGeometry  BasedOnType=Mass  Density=7986.89  DensityUnits=kg/m^3  Mass=680.695  MassUnits=g  CenterOfMass=[0.00, 0.00, 7.613]  CenterOfMassUnits=mm  MomentsOfInertia=[1 1 1]  MomentsOfInertiaUnits=g*mm^2  ProductsOfInertia=[0 0 0]  ProductsOfInertiaUnits=g*mm^2  GraphicType=FromGeometry  MarkerShape=Sphere  MarkerSize=10  GraphicVisPropType=SimpleVisualProperties  GraphicDiffuseColor=[0.5 0.5 0.5]  GraphicOpacity=1.0  GraphicSpecularColor=[0.5 0.5 0.5 1.0]  GraphicAmbientColor=[0.15 0.15 0.15 1.0]  GraphicEmissiveColor=[0.0 0.0 0.0 1.0]  GraphicShininess=75  DoExposeReferenceFrame=on  SerializedFrames=<Frames/>
  joint 1 : PMIOPort  Side=Left
  joint 2 : PMIOPort  Port=2  Side=Right
  connections:
  OriginTransform revolute link_3/LConn1 -- joint 1/RConn1 -- Reference Frame/RConn1 -- link_2/RConn1
  AxisTransform revolute link_3/LConn1 -- OriginTransform revolute link_3/RConn1
  joint 2/RConn1 -- AxisTransform revolute link_3/RConn1

== system Firmware/Plant/Arm/link_3 ==
  AxisTransform revolute link_4 : sm_lib/Frames and Transforms/Rigid Transform  RotationMethod=StandardAxis  FollAlignAxisA=+X  BaseAlignAxisA=+Y  FollAlignAxisB=+Y  BaseAlignAxisB=+Z  RotationStandardAxis=+X  RotationAngle=180  RotationAngleUnits=deg  RotationArbitraryAxis=[0 0 1]  RotationSequenceAxes=FollowerAxes  RotationSequence=XYZ  RotationSequenceAngles=[0 0 119.162]  RotationSequenceAnglesUnits=deg  RotationMatrix=[0 0 0; 0 0 0; 0 0 0]  Quaternion=[1 0 0 0]  TranslationMethod=None  TranslationCartesianOffset=[0 0 0]  TranslationCartesianOffsetUnits=m  TranslationStandardAxis=+Z  TranslationStandardOffset=0  TranslationStandardOffsetUnits=m  TranslationROffset=0  TranslationROffsetUnits=m  TranslationThetaOffset=0  TranslationThetaOffsetUnits=deg  TranslationZOffset=0  TranslationZOffsetUnits=m
  OriginTransform revolute link_4 : sm_lib/Frames and Transforms/Rigid Transform  RotationMethod=None  FollAlignAxisA=+X  BaseAlignAxisA=+Y  FollAlignAxisB=+Y  BaseAlignAxisB=+Z  RotationStandardAxis=+Z  RotationAngle=0  RotationAngleUnits=deg  RotationArbitraryAxis=[0 0 1]  RotationSequenceAxes=FollowerAxes  RotationSequence=XYX  RotationSequenceAngles=[0 0 0]  RotationSequenceAnglesUnits=deg  RotationMatrix=[1 0 0;0 1 0;0 0 1]  Quaternion=[1 0 0 0]  TranslationMethod=Cartesian  TranslationCartesianOffset=[165.60 0.00 48.657]  TranslationCartesianOffsetUnits=mm  TranslationStandardAxis=+Z  TranslationStandardOffset=0  TranslationStandardOffsetUnits=m  TranslationROffset=0  TranslationROffsetUnits=m  TranslationThetaOffset=0  TranslationThetaOffsetUnits=deg  TranslationZOffset=0  TranslationZOffsetUnits=m
  Reference Frame : sm_lib/Frames and Transforms/Reference Frame
  link_3 : sm_lib/Body Elements/File Solid  ExtGeomFileName=./meshes/link_3.stl  UnitType=Custom  ExtGeomFileUnits=mm  StepReaderType=HEX  ExportConvexHullGeometry=off  InertiaType=CalculateFromGeometry  BasedOnType=Mass  Density=7986.89  DensityUnits=kg/m^3  Mass=680.695  MassUnits=g  CenterOfMass=[0.00, 0.00, 7.613]  CenterOfMassUnits=mm  MomentsOfInertia=[1 1 1]  MomentsOfInertiaUnits=g*mm^2  ProductsOfInertia=[0 0 0]  ProductsOfInertiaUnits=g*mm^2  GraphicType=FromGeometry  MarkerShape=Sphere  MarkerSize=10  GraphicVisPropType=SimpleVisualProperties  GraphicDiffuseColor=[0.5 0.5 0.5]  GraphicOpacity=1.0  GraphicSpecularColor=[0.5 0.5 0.5 1.0]  GraphicAmbientColor=[0.15 0.15 0.15 1.0]  GraphicEmissiveColor=[0.0 0.0 0.0 1.0]  GraphicShininess=75  DoExposeReferenceFrame=on  SerializedFrames=<Frames/>
  joint 2 : PMIOPort  Side=Left
  joint 3 : PMIOPort  Port=2  Side=Right
  connections:
  OriginTransform revolute link_4/LConn1 -- joint 2/RConn1 -- Reference Frame/RConn1 -- link_3/RConn1
  AxisTransform revolute link_4/LConn1 -- OriginTransform revolute link_4/RConn1
  joint 3/RConn1 -- AxisTransform revolute link_4/RConn1
